simulink model "transmission_model_v2"  (R2022b)
settings: Solver=ode45  StartTime=0.0  StopTime=6/60  RelTol=1e-3  EnableMultiTasking=on
libraries: spsGroundLib x2, spsThreePhaseProgrammableVoltageSourceLib x2, spsThreePhaseSeriesRLCBranchLib x2, spsThreePhasePISectionLineLib x2, spsThreePhaseVIMeasurementLib x2, spsThreePhaseFaultLib x1, spsThreePhaseSeriesRLCLoadLib x1, spspowerguiLib x1
settings Model: Creator=iyasi  LastModifiedBy=iyasi
settings SolverCC: AlgebraicLoopSolver=TrustRegion
settings DataIOCC: LimitDataPoints=on  SaveFormat=Array
settings OptimizationCC: LifeSpan=inf
settings DebuggingCC: UnconnectedInputMsg=warning  UnconnectedOutputMsg=warning  UnconnectedLineMsg=warning  SFUnexpectedBacktrackingDiag=warning  SFNoUnconditionalDefaultTransitionDiag=warning  SFExecutionAtInitializationDiag=none  SFMachineParentedDataDiag=warning  ArithmeticOperatorsInVariantConditions=warning
settings HardwareCC: ProdBitPerPointer=32  ProdBitPerSizeT=32  ProdBitPerPtrDiffT=32  ProdLargestAtomicFloat=None  ProdIntDivRoundTo=Undefined  ProdEndianess=Unspecified  ProdWordSize=32  ProdHWDeviceType=32-bit Generic
settings ModelReferenceCC: PropagateSignalLabelsOutOfModel=off
settings SFSimCC: SimUseLocalCustomCode=off  CustomCodeUndefinedFunction=UseInterfaceOnly
settings RTWCC: RTWUseLocalCustomCode=off
settings CodeAppCC: StateflowObjectComments=on
settings GRTTargetCC: TargetLangStandard=C89/C90 (ANSI)
settings ConfigComp: CovMetricSettings=dw  CovSaveCumulativeToWorkspaceVar=on  CovSaveSingleToWorkspaceVar=on  CovExternalEMLEnable=off
settings SimscapeCC: SimscapeNormalizeSystem=off

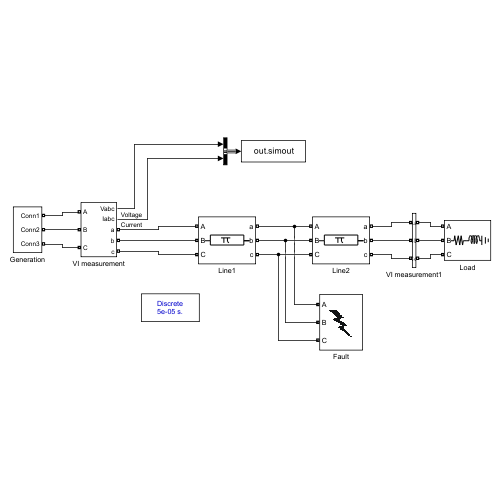
[thumbnail: Simulink's stored preview of the top-level diagram]
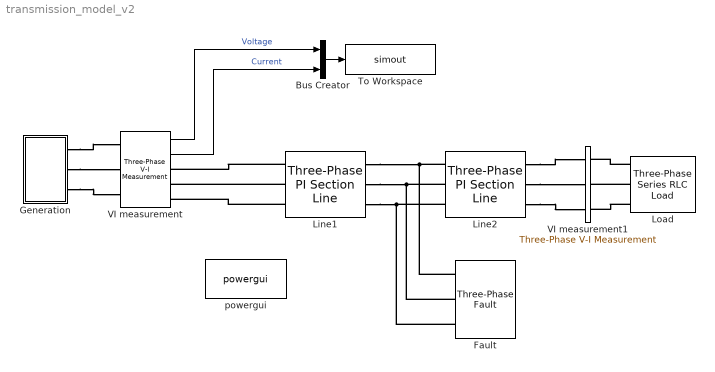
== system transmission_model_v2 ==
  Bus Creator : BusCreator  Inputs=2
  Fault : spsThreePhaseFaultLib/Three-Phase Fault  InitialStates=0  FaultA=on  FaultB=off  FaultC=on  GroundFault=on  SwitchTimes=[0.066638 1.0]  External=off  SwitchStatus=NaN  FaultResistance=0.053205  GroundResistance=10e-10  SnubberResistance=1e6  SnubberCapacitance=inf  Measurements=None
  Generation : Subsystem
  Line1 : spsThreePhasePISectionLineLib/Three-Phase PI Section Line  LConnTagsString=a|b|c  RConnTagsString=A|B|C  Length=47.5034  Frequency=60  Resistances=[ 0.0243 0.3167]  Inductances="[ 0.9238e-3  3.2220e-3]"  Capacitances=[0.0126e-6 0.0078e-6]
  Line2 : spsThreePhasePISectionLineLib/Three-Phase PI Section Line  LConnTagsString=a|b|c  RConnTagsString=A|B|C  Length=252.4966  Frequency=60  Resistances=[ 0.0243 0.3167]  Inductances="[ 0.9238e-3  3.2220e-3]"  Capacitances=[0.0126e-6 0.0078e-6]
  Load : spsThreePhaseSeriesRLCLoadLib/Three-Phase Series RLC Load  LConnTagsString=A|B|C  Configuration=Y (grounded)  NominalVoltage=230e3  Vabc=[1e3 1e3 1e3]  Vabcp=[1e3 1e3 1e3]  NominalFrequency=60  UnbalancedPower=off  ActivePower=200e6  InductivePower=75e6  CapacitivePower=0  Pabc=[10e3 9e3 11e3]  QLabc=[100 90 110]  QCabc=[100 90 110]  Pabcp=[10e3 9e3 11e3]  QLabcp=[100 90 110]  QCabcp=[100 90 110]  Measurements=None  LoadType=constant PQ
  To Workspace : ToWorkspace  VariableName=simout  SaveFormat=Structure With Time  SampleTime=-1
  VI measurement : spsThreePhaseVIMeasurementLib/Three-Phase V-I Measurement  VoltageMeasurement=phase-to-ground  SetLabelV=off  LabelV=Vabc  Vpu=on  VpuLL=off  CurrentMeasurement=yes  SetLabelI=off  LabelI=Iabc  Ipu=on  Pbase=100e6  Vbase=230e3  OutputType=Complex  PhasorSimulation=off  PSBequivalent=0
  VI measurement1 : spsThreePhaseVIMeasurementLib/Three-Phase V-I Measurement  VoltageMeasurement=no  SetLabelV=off  LabelV=Vabc  Vpu=on  VpuLL=off  CurrentMeasurement=no  SetLabelI=off  LabelI=Iabc  Ipu=on  Pbase=100e6  Vbase=230e3  OutputType=Complex  PhasorSimulation=off  PSBequivalent=0
  powergui : spspowerguiLib/powergui  Priority=1  SimulationMode=Discrete  SampleTime=50e-6  frequency=60  Iterations=50  frequencyindice=60  Pbase=100e6  ErrMax=1e-4  UnitsV=kV  UnitsW=MW  buscounter=0  FunctionMessages=off  echomessages=off  EnableUseOfTLC=off  CurrentSourceSwitches=off  DisableSnubberDevices=off  DisableRonSwitches=off  DisableVfSwitches=off  DisplayEquations=off  AutomaticDiscreteSolvers=off  SolverType=Tustin/Backward Euler (TBE)  Interpol=off  ExternalGateDelay=off  methode=off  Ts=100  x0status=blocks  SPID=on  SwTol=0  HookPort=off  NonlinearTolerance=1e-4  nMaxIteration=100  ContinueOnMaxIteration=off  RestoreLinks=warning  ResistiveCurrentMeasurement=off  Frange=[0:2:500]  Ylog=off  Xlog=on  ShowGrid=off  save=off  variable=ZData  structure=0  ZoomFFT=off  StartTime=0.0  cycles=1  DisplayStyle=1  fundamental=60  FreqAxis=off  MaxFrequency=1000  frequencyindicesteady=1  RmsSteady=1  display=off
  wires:
  VI measurement/1 -> Bus Creator/1  "Voltage"
  VI measurement/2 -> Bus Creator/2  "Current"
  Bus Creator/1 -> To Workspace/1
  connections:
  Line1/LConn1 -- VI measurement/RConn1
  Line1/LConn2 -- VI measurement/RConn2
  Line1/LConn3 -- VI measurement/RConn3
  Line1/RConn1 -- Line2/LConn1 -- Fault/LConn1
  Line1/RConn2 -- Line2/LConn2 -- Fault/LConn2
  Line1/RConn3 -- Line2/LConn3 -- Fault/LConn3
  Line2/RConn2 -- VI measurement1/RConn2
  Load/LConn2 -- VI measurement1/LConn2
  Load/LConn1 -- VI measurement1/LConn1
  Load/LConn3 -- VI measurement1/LConn3
  Line2/RConn1 -- VI measurement1/RConn1
  Line2/RConn3 -- VI measurement1/RConn3
  Generation/RConn1 -- VI measurement/LConn1
  Generation/RConn2 -- VI measurement/LConn2
  Generation/RConn3 -- VI measurement/LConn3

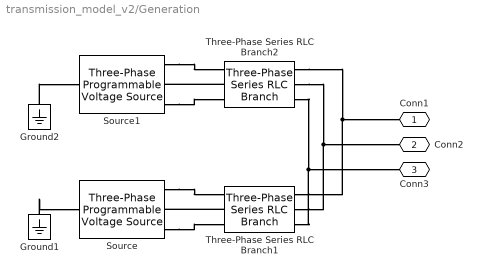
== system transmission_model_v2/Generation ==
  Ground1 : spsGroundLib/Ground  LConnTagsString=a
  Ground2 : spsGroundLib/Ground  LConnTagsString=a
  Source : spsThreePhaseProgrammableVoltageSourceLib/Three-Phase Programmable Voltage Source  PositiveSequence="[230e3  0 60]"  VariationEntity=None  VariationType=Table of time-amplitude pairs  VariationTypeAlt=Step  VariationStep=0.5  VariationRate=10  VariationMagnitude=0.3  VariationFrequency=2  VariationTiming=[1 2]  VariationPhaseA=off  Amplitudes=[1 0.8 1.2 1.0]  TimeValues=[0 0.1 0.15 0.2]  HarmonicGeneration=off  HarmonicA=[3 0.044036056222235 260.287227517709 0]  HarmonicB=[5 0.0176427166594859 84.7302203099656 2]  Timing="[0  1]"  BusType=swing  Pref=0  Qref=0  Qmin=-inf  Qmax=inf
  Source1 : spsThreePhaseProgrammableVoltageSourceLib/Three-Phase Programmable Voltage Source  PositiveSequence="[230e3  0 60]"  VariationEntity=None  VariationType=Table of time-amplitude pairs  VariationTypeAlt=Step  VariationStep=0.5  VariationRate=10  VariationMagnitude=0.3  VariationFrequency=2  VariationTiming=[1 2]  VariationPhaseA=off  Amplitudes=[1 0.8 1.2 1.0]  TimeValues=[0 0.1 0.15 0.2]  HarmonicGeneration=on  HarmonicA=[7 0.0350232556018142 157.218872830535 1]  HarmonicB=[11 0.0229672937384309 231.822019462207 2]  Timing="[0  1]"  BusType=swing  Pref=0  Qref=0  Qmin=-inf  Qmax=inf
  Three-Phase Series RLC Branch1 : spsThreePhaseSeriesRLCBranchLib/Three-Phase Series RLC Branch  LConnTagsString=A|B|C  RConnTagsString=A|B|C  BranchType=RL  Resistance=0.8929  Inductance=16.58e-3  Capacitance=1e-6  Measurements=None
  Three-Phase Series RLC Branch2 : spsThreePhaseSeriesRLCBranchLib/Three-Phase Series RLC Branch  LConnTagsString=A|B|C  RConnTagsString=A|B|C  BranchType=RL  Resistance=0.8929  Inductance=16.58e-3  Capacitance=1e-6  Measurements=None
  Conn1 : PMIOPort  Side=Right
  Conn2 : PMIOPort  Port=2  Side=Right
  Conn3 : PMIOPort  Port=3  Side=Right
  connections:
  Source/RConn1 -- Three-Phase Series RLC Branch1/LConn1
  Three-Phase Series RLC Branch1/RConn3 -- Conn3/RConn1 -- Three-Phase Series RLC Branch2/RConn3
  Three-Phase Series RLC Branch2/LConn2 -- Source1/RConn2
  Three-Phase Series RLC Branch1/RConn2 -- Conn2/RConn1 -- Three-Phase Series RLC Branch2/RConn2
  Ground1/LConn1 -- Source/LConn1
  Ground2/LConn1 -- Source1/LConn1
  Source/RConn3 -- Three-Phase Series RLC Branch1/LConn3
  Source1/RConn1 -- Three-Phase Series RLC Branch2/LConn1
  Source1/RConn3 -- Three-Phase Series RLC Branch2/LConn3
  Three-Phase Series RLC Branch1/RConn1 -- Conn1/RConn1 -- Three-Phase Series RLC Branch2/RConn1
  Three-Phase Series RLC Branch1/LConn2 -- Source/RConn2
